simulink model "Stage4_PLL_STNF_K60"  (R2024b)
settings: Solver=ode1  StartTime=0.0  StopTime=2  FixedStep=Ts  RelTol=1e-3
InitFcn:
  | %% ===== Global =====
  | Ts = 1e-6;                        % pas d'echantillonnage [s]
  | 
  | %% ===== PV (module 550 W, rapport) =====
  | Nser = 14;  Npar = 4;
  | % Donnees du module : recopiees EN DUR dans le bloc PV Array
  | % (le masque n'accepte pas de variables dans Module data)
  | Ncell_mod = 144;
  | Voc_mod = 49.80;  Isc_mod = 13.98;
  | Vm_mod  = 41.95;  Im_mod  = 13.12;
  | kVoc = -0.270;    kIsc = 0.048;   % [%/deg.C]
  | C_pv = 470e-6;                    % condensateur PV [F]
  | 
  | %% ===== Profil d'eclairement =====
  | G1     = 1000;                    % [W/m2] avant l'echelon
  | G2     = 700;                     % [W/m2] apres l'echelon
  | t_step = 1;                       % [s] instant de l'echelon
  | 
  | %% ===== Boost PV =====
  | L_boost = 7.97e-3;                % [H]
  | C_dc    = 3e-3;                   % [F] condensateur du bus
  | fsw_dc  = 10e3;                   % [Hz]
  | D_test  = 0.344;                  % D fixe (etape 3.0, bloc commente)
  | R_dc    = 26;                     % [ohm] (etape 3.0, non utilise)
  | 
  | %% ===== MPPT IncCond =====
  | T_mppt = 20e-3;   % periode MPPT [s]
  | dD     = 0.005;                   % pas de perturbation
  | D0     = 0.25;                    % > 1 - Voc/V_ref = 0.23
  | D_min  = 0.05;
  | D_max  = 0.9;
  | 
  | %% ===== Filtre anti-repliement des mesures MPPT =====
  | tau_f = 0.5e-3;                   % [s]
  | a_f   = exp(-Ts/tau_f);
  | 
  | %% ===== Bus DC fixe (etape 3, retire a l'etape 4.3) =====
  | V_bus = 900;                      % [V]
  | R_bus = 0.1;                      % [ohm]
  | 
  | %% ===== Batterie (Etape 4) =====
  | V_bat_nom = 196;                  % [V] tension nominale NiMH
  | Q_bat     = 150;                  % [Ah] capacite
  | SOC0      = 80;                   % [%] etat de charge initial
  | 
  | %% ===== Hacheur bidirectionnel =====
  | L_bat     = 3e-3;                 % [H] redimensionnee (au lieu de 5 H)
  | fsw_bat   = 10e3;                 % [Hz]
  | I_bat_max = 30;                   % [A] saturation de la reference
  | 
  | %% ===== Boucle de courant (interne) : fc ~ 1 kHz =====
  | Kp_i = 0.021;                     % = wc*L_bat/V_ref
  | Ki_i = 26;                        % zero a wc/5
  | 
  | %% ===== Boucle de tension du bus (externe) : fc ~ 50 Hz =====
  | V_ref = 900;                      % [V]
  | Kp_v  = 4.3;                      % = wc*C_dc/(1-D), D = 1 - V_bat/V_ref
  | Ki_v  = 270;                      % zero a wc/5
  | 
  | %% ===== Charge DC =====
  | ... (+96 lines)
undefined symbols (not defined in the file or in its folder): DiscIntNeverNeededParam, dspblkCoreblockFVToolHelper, gcbh, Hydride, Metal, Nickel, sgn
libraries: slpidlib x5, spsSeriesRLCBranchLib x3, spsVoltageMeasurementLib x3, spsUniversalBridgeLib x2, spsPWMGeneratorDCDCLib x2, spsabctodq0Lib x2, spsCurrentMeasurementLib x2, spsThreePhaseSeriesRLCBranchLib x2, spsBatteryLib x1, spsParallelRLCBranchLib x1, spsdq0toabcLib x1, spsPVArrayLib x1
(part 2 of 2)

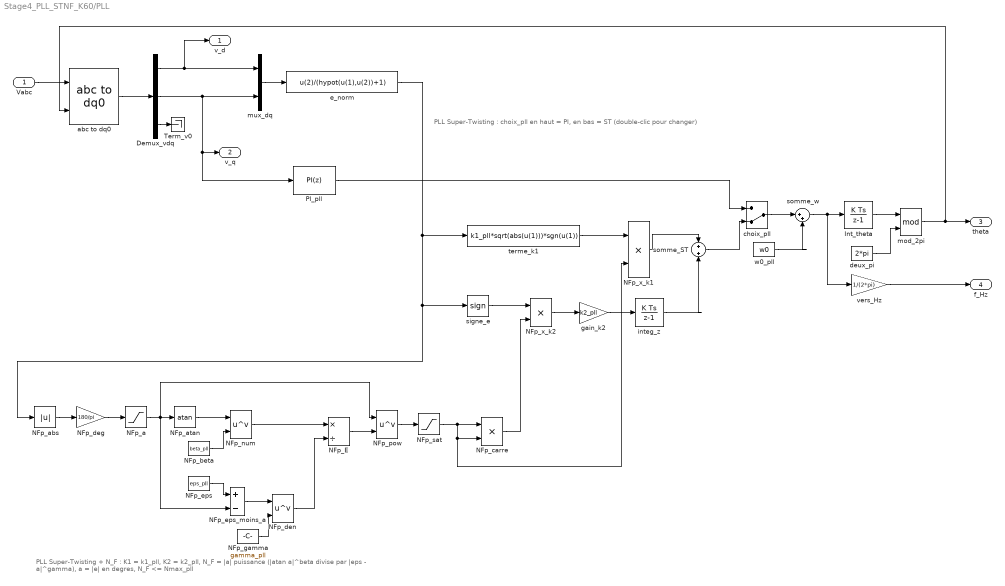
== system Stage4_PLL_STNF_K60/PLL ==
  note: PLL Super-Twisting : choix_pll en haut = PI, en bas = ST (double-clic pour changer)
  note: PLL Super-Twisting + N_F : K1 = k1_pll, K2 = k2_pll, N_F = |a| puissance (|atan a|^beta divise par |eps - a|^gamma), a = |e| en degres, N_F <= Nmax_pll
  Vabc : Inport
  Demux_vdq : Demux  Outputs=3
  Int_theta : DiscreteIntegrator  gainval=1  SampleTime=Ts  ICPrevOutput=DiscIntNeverNeededParam  ICPrevScaledInput=DiscIntNeverNeededParam
  NFp_E : Product  Inputs=*/
  NFp_a : Saturate  UpperLimit=0.99*eps_pll  LowerLimit=0
  NFp_abs : Abs  SaturateOnIntegerOverflow=off
  NFp_atan : Trigonometry  Operator=atan
  NFp_beta : Constant  Value=beta_pll
  NFp_carre : Product
  NFp_deg : Gain  Gain=180/pi
  NFp_den : Math  Operator=pow
  NFp_eps : Constant  Value=eps_pll
  NFp_eps_moins_a : Sum  Inputs=+-
  NFp_gamma : Constant  Value=gamma_pll
  NFp_num : Math  Operator=pow
  NFp_pow : Math  Operator=pow
  NFp_sat : Saturate  UpperLimit=Nmax_pll  LowerLimit=0
  NFp_x_k1 : Product
  NFp_x_k2 : Product
  PI_pll : slpidlib/PID Controller  Controller=PI  Form=Parallel  TimeDomain=Discrete-time  UseExternalTs=off  SampleTime=Ts  IntegratorMethod=Forward Euler  FilterMethod=Forward Euler  ControllerParametersSource=internal  P=Kp_pll  I=Ki_pll  UseKiTs=off  D=0  UseExternalDerivativeSource=off  N=100  UseFilter=on  TunerSelectOption=Transfer Function Based (PID Tuner App)  InitialConditionSource=internal  InitialConditionForIntegrator=0  InitialConditionForFilter=0  DifferentiatorICPrevScaledInput=0  ExternalReset=none  TrackingMode=off  Kt=1  LimitOutput=on  SatLimitsSource=internal  UpperSaturationLimit=dw_max  LowerSaturationLimit=-dw_max  LinearizeAsGain=on  AntiWindupMode=clamping  Kb=1  LimitIntegrator=off  UpperIntegratorSaturationLimit=inf  LowerIntegratorSaturationLimit=-inf  POutMin=[]  POutMax=[]  IOutMin=[]  IOutMax=[]  DOutMin=[]  DOutMax=[]  NOutMin=[]  NOutMax=[]  SumOutMin=[]  SumOutMax=[]  SaturationOutMin=[]  SaturationOutMax=[]  PParamMin=[]  PParamMax=[]  IParamMin=[]  IParamMax=[]  DParamMin=[]  DParamMax=[]  NParamMin=[]  NParamMax=[]  KbParamMin=[]  KbParamMax=[]  KtParamMin=[]  KtParamMax=[]  KbOutMin=[]  KbOutMax=[]  KtOutMin=[]  KtOutMax=[]  IntegratorOutMin=[]  IntegratorOutMax=[]  FilterOutMin=[]  FilterOutMax=[]  SumI1OutMin=[]  SumI1OutMax=[]  SumI2OutMin=[]  SumI2OutMax=[]  SumI3OutMin=[]  SumI3OutMax=[]  SumI4OutMin=[]  SumI4OutMax=[]  SumDOutMin=[]  SumDOutMax=[]  DifferentiatorOutMin=[]  DifferentiatorOutMax=[]  FilterDiffOutCoefMin=[]  FilterDiffOutCoefMax=[]  ReciprocalOutMin=[]  ReciprocalOutMax=[]  SumDenOutMin=[]  SumDenOutMax=[]  SumNumOutMin=[]  SumNumOutMax=[]  DivideOutMin=[]  DivideOutMax=[]  UdiffTsProdOutMin=[]  UdiffTsProdOutMax=[]  NTsProdOutMin=[]  NTsProdOutMax=[]  UintegralTsProdOutMin=[]  UintegralTsProdOutMax=[]  UngainTsProdOutMin=[]  UngainTsProdOutMax=[]  ClampingZeroOutDataTypeStr=Inherit: Inherit via back propagation  ClampingZeroOutMin=[]  ClampingZeroOutMax=[]  FilterDenConstantOutDataTypeStr=Inherit: Inherit via back propagation  FilterDenConstantOutMin=[]  FilterDenConstantOutMax=[]  PCopyOutDataTypeStr=Inherit: Inherit via back propagation  PCopyOutMin=[]  PCopyOutMax=[]  NCopyOutDataTypeStr=Inherit: Inherit via back propagation  NCopyOutMin=[]  NCopyOutMax=[]  IntegratorContinuousStateAttributes=''  IntegratorStateMustResolveToSignalObject=off  IntegratorRTWStateStorageClass=Auto  FilterContinuousStateAttributes=''  FilterStateMustResolveToSignalObject=off  FilterRTWStateStorageClass=Auto  ParallelPVariant=InternalParameters  IdealPVariant=Disabled  IVariant=InternalParameters  DVariant=Disabled  IntegratorVariant=Discrete  SatVariant=Enabled  AWVariant=DiscClampingParallel  PCopyVariant=Disabled  TRVariant=Disabled  FdbkBlocksVariant=Forward  IdealPFdbkVariant=Disabled  SatFdbkVariant=Disabled  DerivativeFilterVariant=Disabled  NVariant=Disabled  NCopyVariant=Disabled_SignalSpec  FilterICVariant=Disabled  IntegratorICVariant=InternalICs  ExternalResetVariant=Disabled  TRSumVariant=Passthrough  SumFdbkVariant=Disabled  SumVariant=Sum_PI  TsampFilterVariant=InternalTs  TsampNgainVariant=Passthrough  TsampIntegralVariant=Disabled_SignalSpec  ExternalSaturationOutDataTypeStr=Inherit: Same as second input  DerivativeSourceVariant=Disabled  PreIntVariant=InternalPreInt
      settings: LibrarySourceBlock=simulink/Discrete/Discrete PID Controller
  Term_v0 : Terminator
  abc to dq0 : spsabctodq0Lib/abc to dq0  Alignment=90 degrees behind phase A axis
  choix_pll : ManualSwitch  CurrentSetting=0
  deux_pi : Constant  Value=2*pi
  e_norm : Fcn  Expr=u(2)/(hypot(u(1),u(2))+1)
  gain_k2 : Gain  Gain=k2_pll
  integ_z : DiscreteIntegrator  SampleTime=Ts  ICPrevOutput=DiscIntNeverNeededParam  ICPrevScaledInput=DiscIntNeverNeededParam
  mod_2pi : Math  Operator=mod
  mux_dq : Mux  Inputs=2
  signe_e : Signum
  somme_ST : Sum
  somme_w : Sum  Inputs=|++
  terme_k1 : Fcn  Expr=k1_pll*sqrt(abs(u(1)))*sgn(u(1))
  vers_Hz : Gain  Gain=1/(2*pi)
  w0_pll : Constant  Value=w0
  v_d : Outport
  v_q : Outport  Port=2
  theta : Outport  Port=3
  f_Hz : Outport  Port=4
  wires:
  Vabc/1 -> abc to dq0/1
  abc to dq0/1 -> Demux_vdq/1
  Demux_vdq/1 -> mux_dq/1, v_d/1
  Demux_vdq/2 -> mux_dq/2, v_q/1, PI_pll/1
  Demux_vdq/3 -> Term_v0/1
  mux_dq/1 -> e_norm/1
  e_norm/1 -> terme_k1/1, signe_e/1, NFp_abs/1
  PI_pll/1 -> choix_pll/1
  terme_k1/1 -> NFp_x_k1/1
  NFp_x_k1/1 -> somme_ST/1
  signe_e/1 -> NFp_x_k2/1
  NFp_x_k2/1 -> gain_k2/1
  gain_k2/1 -> integ_z/1
  integ_z/1 -> somme_ST/2
  somme_ST/1 -> choix_pll/2
  choix_pll/1 -> somme_w/1
  w0_pll/1 -> somme_w/2
  somme_w/1 -> Int_theta/1, vers_Hz/1
  Int_theta/1 -> mod_2pi/1
  deux_pi/1 -> mod_2pi/2
  mod_2pi/1 -> theta/1, abc to dq0/2
  vers_Hz/1 -> f_Hz/1
  NFp_abs/1 -> NFp_deg/1
  NFp_deg/1 -> NFp_a/1
  NFp_a/1 -> NFp_atan/1, NFp_pow/1, NFp_eps_moins_a/2
  NFp_atan/1 -> NFp_num/1
  NFp_beta/1 -> NFp_num/2
  NFp_eps/1 -> NFp_eps_moins_a/1
  NFp_eps_moins_a/1 -> NFp_den/1
  NFp_gamma/1 -> NFp_den/2
  NFp_num/1 -> NFp_E/1
  NFp_den/1 -> NFp_E/2
  NFp_E/1 -> NFp_pow/2
  NFp_pow/1 -> NFp_sat/1
  NFp_sat/1 -> NFp_carre/1, NFp_carre/2, NFp_x_k1/2
  NFp_carre/1 -> NFp_x_k2/2

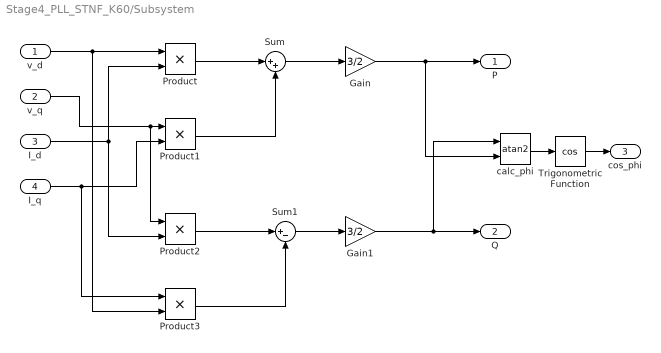
== system Stage4_PLL_STNF_K60/Subsystem ==
  v_d : Inport
  v_q : Inport  Port=2
  I_d : Inport  Port=3
  I_q : Inport  Port=4
  Gain : Gain  Gain=3/2
  Gain1 : Gain  Gain=3/2
  Product{,1..3} (4 alike) : Product
  Sum : Sum  Inputs=|++
  Sum1 : Sum  Inputs=|+-
  Trigonometric Function : Trigonometry  Operator=cos
  calc_phi : Trigonometry  Operator=atan2
  P : Outport
  Q : Outport  Port=2
  cos_phi : Outport  Port=3
  wires:
  v_d/1 -> Product3/2, Product/1
  I_d/1 -> Product2/2, Product/2
  v_q/1 -> Product2/1, Product1/1
  I_q/1 -> Product3/1, Product1/2
  Sum/1 -> Gain/1
  Product/1 -> Sum/1
  Product1/1 -> Sum/2
  Gain/1 -> calc_phi/2, P/1
  Product2/1 -> Sum1/1
  Product3/1 -> Sum1/2
  Sum1/1 -> Gain1/1
  Gain1/1 -> calc_phi/1, Q/1
  calc_phi/1 -> Trigonometric Function/1
  Trigonometric Function/1 -> cos_phi/1

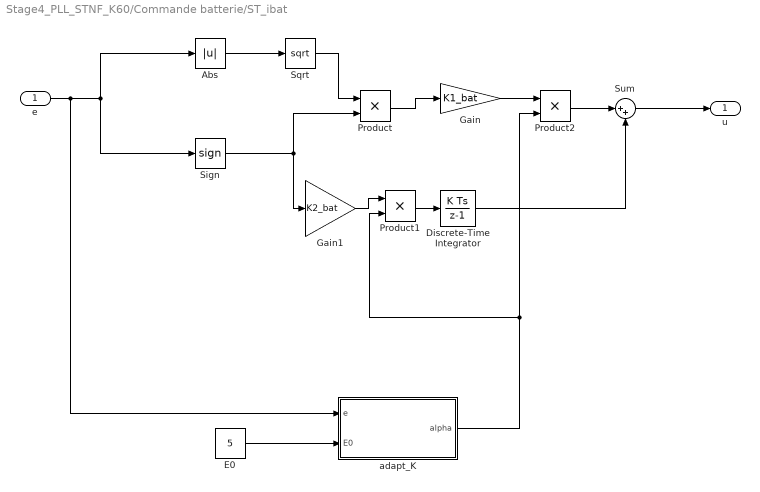
== system Stage4_PLL_STNF_K60/Commande batterie/ST_ibat ==
  e : Inport
  Abs : Abs  SaturateOnIntegerOverflow=off
  Discrete-Time Integrator : DiscreteIntegrator  SampleTime=Ts  ICPrevOutput=DiscIntNeverNeededParam  ICPrevScaledInput=DiscIntNeverNeededParam
  E0 : Constant  Value=5
  Gain : Gain  Gain=K1_bat
  Gain1 : Gain  Gain=K2_bat
  Product : Product
  Product1 : Product
  Product2 : Product
  Sign : Signum
  Sqrt : Sqrt
  Sum : Sum  Inputs=|++
  adapt_K : MATLAB Function  TreatAsAtomicUnit=on  SystemSampleTime=Ts
  u : Outport
  wires:
  e/1 -> adapt_K/1(e), Abs/1, Sign/1
  Abs/1 -> Sqrt/1
  Sqrt/1 -> Product/1
  Sign/1 -> Product/2, Gain1/1
  Product/1 -> Gain/1
  Discrete-Time Integrator/1 -> Sum/2
  Sum/1 -> u/1
  E0/1 -> adapt_K/2(E0)
  Gain/1 -> Product2/1
  adapt_K/1(alpha) -> Product1/2, Product2/2
  Gain1/1 -> Product1/1
  Product1/1 -> Discrete-Time Integrator/1
  Product2/1 -> Sum/1

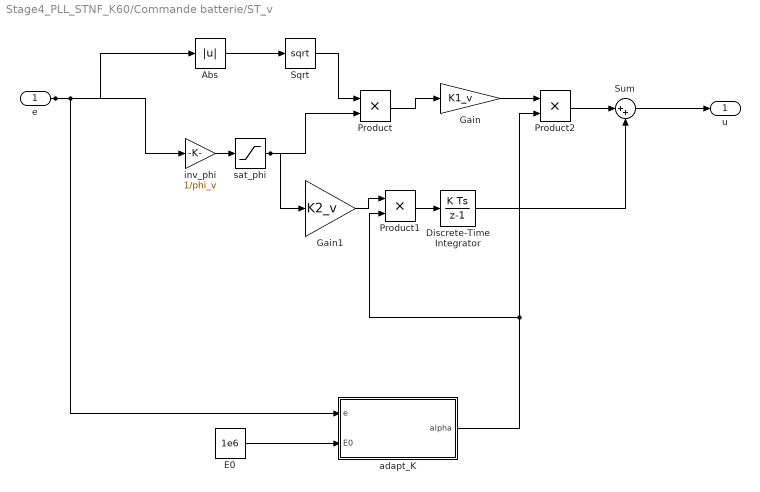
== system Stage4_PLL_STNF_K60/Commande batterie/ST_v ==
  e : Inport
  Abs : Abs  SaturateOnIntegerOverflow=off
  Discrete-Time Integrator : DiscreteIntegrator  SampleTime=Ts  ICPrevOutput=DiscIntNeverNeededParam  ICPrevScaledInput=DiscIntNeverNeededParam
  E0 : Constant  Value=1e6
  Gain : Gain  Gain=K1_v
  Gain1 : Gain  Gain=K2_v
  Product : Product
  Product1 : Product
  Product2 : Product
  Sqrt : Sqrt
  Sum : Sum  Inputs=|++
  adapt_K : MATLAB Function  TreatAsAtomicUnit=on  SystemSampleTime=Ts
  inv_phi : Gain  Gain=1/phi_v
  sat_phi : Saturate  UpperLimit=1  LowerLimit=-1
  u : Outport
  wires:
  Product2/1 -> Sum/1
  Product1/1 -> Discrete-Time Integrator/1
  Gain1/1 -> Product1/1
  adapt_K/1(alpha) -> Product2/2, Product1/2
  Gain/1 -> Product2/1
  E0/1 -> adapt_K/2(E0)
  Sum/1 -> u/1
  Discrete-Time Integrator/1 -> Sum/2
  Product/1 -> Gain/1
  Sqrt/1 -> Product/1
  Abs/1 -> Sqrt/1
  e/1 -> adapt_K/1(e), Abs/1, inv_phi/1
  inv_phi/1 -> sat_phi/1
  sat_phi/1 -> Gain1/1, Product/2

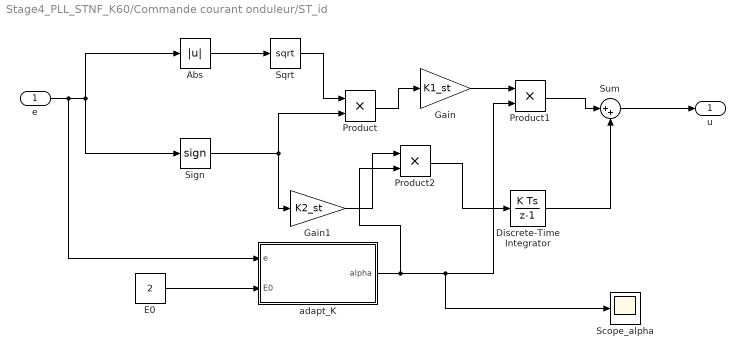
== system Stage4_PLL_STNF_K60/Commande courant onduleur/ST_id ==
  e : Inport
  Abs : Abs  SaturateOnIntegerOverflow=off
  Discrete-Time Integrator : DiscreteIntegrator  SampleTime=Ts  ICPrevOutput=DiscIntNeverNeededParam  ICPrevScaledInput=DiscIntNeverNeededParam
  E0 : Constant  Value=2
  Gain : Gain  Gain=K1_st
  Gain1 : Gain  Gain=K2_st
  Product : Product
  Product1 : Product
  Product2 : Product
  Scope_alpha : Scope
  Sign : Signum
  Sqrt : Sqrt
  Sum : Sum  Inputs=|++
  adapt_K : MATLAB Function  TreatAsAtomicUnit=on  SystemSampleTime=Ts
  u : Outport
  wires:
  e/1 -> adapt_K/1(e), Abs/1, Sign/1
  Abs/1 -> Sqrt/1
  Sqrt/1 -> Product/1
  Sign/1 -> Product/2, Gain1/1
  Product/1 -> Gain/1
  Discrete-Time Integrator/1 -> Sum/2
  Sum/1 -> u/1
  E0/1 -> adapt_K/2(E0)
  Gain/1 -> Product1/1
  adapt_K/1(alpha) -> Product2/2, Scope_alpha/1, Product1/2
  Product1/1 -> Sum/1
  Gain1/1 -> Product2/1
  Product2/1 -> Discrete-Time Integrator/1

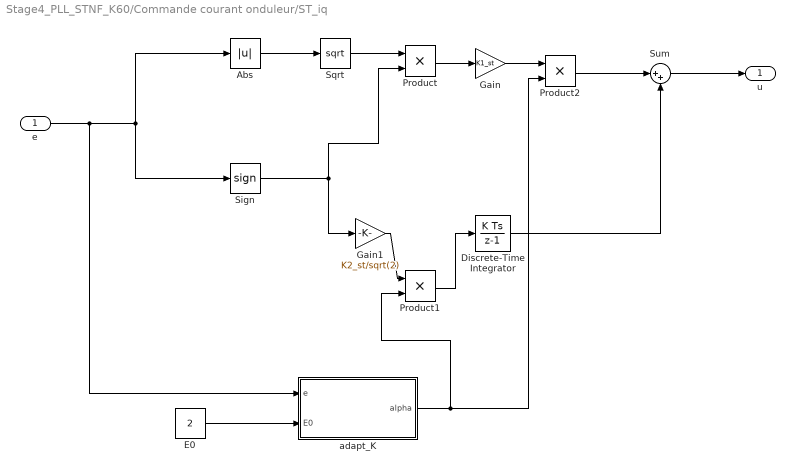
== system Stage4_PLL_STNF_K60/Commande courant onduleur/ST_iq ==
  e : Inport
  Abs : Abs  SaturateOnIntegerOverflow=off
  Discrete-Time Integrator : DiscreteIntegrator  SampleTime=Ts  ICPrevOutput=DiscIntNeverNeededParam  ICPrevScaledInput=DiscIntNeverNeededParam
  E0 : Constant  Value=2
  Gain : Gain  Gain=K1_st
  Gain1 : Gain  Gain=K2_st/sqrt(2)
  Product : Product
  Product1 : Product
  Product2 : Product
  Sign : Signum
  Sqrt : Sqrt
  Sum : Sum  Inputs=|++
  adapt_K : MATLAB Function  TreatAsAtomicUnit=on  SystemSampleTime=Ts
  u : Outport
  wires:
  e/1 -> adapt_K/1(e), Abs/1, Sign/1
  Abs/1 -> Sqrt/1
  Sqrt/1 -> Product/1
  Sign/1 -> Product/2, Gain1/1
  Product/1 -> Gain/1
  Discrete-Time Integrator/1 -> Sum/2
  Sum/1 -> u/1
  E0/1 -> adapt_K/2(E0)
  Gain/1 -> Product2/1
  adapt_K/1(alpha) -> Product1/2, Product2/2
  Gain1/1 -> Product1/1
  Product1/1 -> Discrete-Time Integrator/1
  Product2/1 -> Sum/1

== system Stage4_PLL_STNF_K60/Commande courant onduleur/u_eq_d ==
  v_d : Inport
  I_d : Inport  Port=2
  I_q : Inport  Port=3
  filtre_vd : DiscreteTransferFcn  LoadFcn=dspblkCoreblockFVToolHelper(gcbh,'load');  Numerator=[1-a_ff]  Denominator=[1 -a_ff]  InitialStates=Ts
      settings: CopyFcn=dspblkCoreblockFVToolHelper(gcbh,'copy');  DeleteFcn=dspblkCoreblockFVToolHelper(gcbh,'close');  ModelCloseFcn=dspblkCoreblockFVToolHelper(gcbh,'close');  PreSaveFcn=dspblkCoreblockFVToolHelper(gcbh,'presave');  PostSaveFcn=dspblkCoreblockFVToolHelper(gcbh,'postsave');  CloseFcn=dspblkCoreblockFVToolHelper(gcbh,'close');
  gain_R : Gain  Gain=R_tot
  gain_wL : Gain  Gain=w0*L_tot
  somme_ueq : Sum  Inputs=|++-
  u_eq : Outport
  wires:
  I_d/1 -> gain_R/1
  I_q/1 -> gain_wL/1
  gain_R/1 -> somme_ueq/2
  gain_wL/1 -> somme_ueq/3
  somme_ueq/1 -> u_eq/1
  v_d/1 -> filtre_vd/1
  filtre_vd/1 -> somme_ueq/1

== system Stage4_PLL_STNF_K60/Commande courant onduleur/u_eq_q ==
  vq : Inport
  I_q : Inport  Port=2
  I_d : Inport  Port=3
  filtre_vq : DiscreteTransferFcn  LoadFcn=dspblkCoreblockFVToolHelper(gcbh,'load');  Numerator=[1-a_ff]  Denominator=[1 -a_ff]  InitialStates=Ts
      settings: CopyFcn=dspblkCoreblockFVToolHelper(gcbh,'copy');  DeleteFcn=dspblkCoreblockFVToolHelper(gcbh,'close');  ModelCloseFcn=dspblkCoreblockFVToolHelper(gcbh,'close');  PreSaveFcn=dspblkCoreblockFVToolHelper(gcbh,'presave');  PostSaveFcn=dspblkCoreblockFVToolHelper(gcbh,'postsave');  CloseFcn=dspblkCoreblockFVToolHelper(gcbh,'close');
  gain_R : Gain  Gain=R_tot
  gain_wL : Gain  Gain=w0*L_tot
  somme_ueq : Sum  Inputs=|+++
  u_eq : Outport
  wires:
  I_q/1 -> gain_R/1
  I_d/1 -> gain_wL/1
  gain_R/1 -> somme_ueq/2
  gain_wL/1 -> somme_ueq/3
  somme_ueq/1 -> u_eq/1

== matlab function Stage4_PLL_STNF_K60/Commande courant onduleur/MATLAB Function ==
  data: t input; y output
function y = fcn(t)

if t < 0.5
    y = 4000;

elseif t < 1
    y = 8000;

elseif t < 1.5
    y = 10000;

elseif t < 2
    y = 6000;

else
    y = 6000;
end

end

== matlab function Stage4_PLL_STNF_K60/Commande MPPT/MPPT_IncCond ==
  data: V input; D output; I input; D0 parameter; dD parameter; D_min parameter; D_max parameter
function D = IncCond(V, I, D0, dD, D_min, D_max)
% MPPT conductance incrementale - hacheur Boost
% Boost : Vpv = Vbus(1-D) -> augmenter D fait BAISSER Vpv
persistent V_old I_old D_old
if isempty(V_old)
    V_old = V;  I_old = I;  D_old = D0;
end
dV = V - V_old;
dI = I - I_old;
D  = D_old;

if V > 1
    if I < 0.5                    % PV a vide (Vbus(1-D) > Voc)
        D = D_old + dD;           % baisser Vpv jusqu'a ce que I circule
    elseif dV == 0
        if dI > 0                 % eclairement en hausse -> monter V
            D = D_old - dD;
        elseif dI < 0             % eclairement en baisse -> baisser V
            D = D_old + dD;
        end
    else
        if dI/dV > -I/V           % gauche du MPP -> monter V -> D diminue
            D = D_old - dD;
        elseif dI/dV < -I/V       % droite du MPP -> baisser V -> D augmente
            D = D_old + dD;
        end
    end
end

D = min(max(D, D_min), D_max);    % saturation
V_old = V;  I_old = I;  D_old = D;
end

== matlab function Stage4_PLL_STNF_K60/Commande courant onduleur/ST_id/adapt_K ==
  data: e input; alpha output; E0 input
function alpha = adapt_K(e, E0)
% Adaptation floue des gains du Super-Twisting (Sugeno, 3 regles)
persistent ef
if isempty(ef), ef = 0; end
ef = ef + 0.002*(abs(e) - ef);      % |e| filtre (~0,5 ms) : ignore l'ondulation MLI
x  = ef/E0;                          % erreur normalisee
muP = max(0, 1 - x);                 % Petit : triangle centre en 0
muM = max(0, 1 - abs(x - 1));        % Moyen : triangle centre en 1
muG = min(1, max(0, x - 1));         % Grand : a partir de 2
alpha = (muP*1.0 + muM*1.5 + muG*2.0)/(muP + muM + muG + eps);  % centre de gravite
end

== matlab function Stage4_PLL_STNF_K60/Commande courant onduleur/ST_iq/adapt_K ==
  data: e input; alpha output; E0 input
function alpha = adapt_K(e, E0)
% Adaptation floue des gains du Super-Twisting (Sugeno, 3 regles)
persistent ef
if isempty(ef), ef = 0; end
ef = ef + 0.002*(abs(e) - ef);      % |e| filtre (~0,5 ms) : ignore l'ondulation MLI
x  = ef/E0;                          % erreur normalisee
muP = max(0, 1 - x);                 % Petit : triangle centre en 0
muM = max(0, 1 - abs(x - 1));        % Moyen : triangle centre en 1
muG = min(1, max(0, x - 1));         % Grand : a partir de 2
alpha = (muP*1.0 + muM*1.5 + muG*2.0)/(muP + muM + muG + eps);  % centre de gravite
end

== matlab function Stage4_PLL_STNF_K60/Commande batterie/ST_ibat/adapt_K ==
  data: e input; alpha output; E0 input
function alpha = adapt_K(e, E0)
% Adaptation floue des gains du Super-Twisting (Sugeno, 3 regles)
persistent ef
if isempty(ef), ef = 0; end
ef = ef + 0.002*(abs(e) - ef);      % |e| filtre (~0,5 ms) : ignore l'ondulation MLI
x  = ef/E0;                          % erreur normalisee
muP = max(0, 1 - x);                 % Petit : triangle centre en 0
muM = max(0, 1 - abs(x - 1));        % Moyen : triangle centre en 1
muG = min(1, max(0, x - 1));         % Grand : a partir de 2
alpha = (muP*1.0 + muM*1.5 + muG*2.0)/(muP + muM + muG + eps);  % centre de gravite
end

== matlab function Stage4_PLL_STNF_K60/Commande batterie/ST_v/adapt_K ==
  data: e input; alpha output; E0 input
function alpha = adapt_K(e, E0)
% Adaptation floue des gains du Super-Twisting (Sugeno, 3 regles)
persistent ef
if isempty(ef), ef = 0; end
ef = ef + 0.002*(abs(e) - ef);      % |e| filtre (~0,5 ms) : ignore l'ondulation MLI
x  = ef/E0;                          % erreur normalisee
muP = max(0, 1 - x);                 % Petit : triangle centre en 0
muM = max(0, 1 - abs(x - 1));        % Moyen : triangle centre en 1
muG = min(1, max(0, x - 1));         % Grand : a partir de 2
alpha = (muP*1.0 + muM*1.5 + muG*2.0)/(muP + muM + muG + eps);  % centre de gravite
end
